simulink library "Lib_Piccolo"  (R2018b)
settings: Solver=VariableStepAuto  StartTime=0.0  StopTime=10.0  RelTol=1e-3
values from neighbouring files (symbols this model uses):
  AccelErrInt2Brakes = 0.15    [SimulationControlConfig16P.m]    (also in SimulationControlConfig16P_LEGACY.m; SimulationControlConfigTAILLESS.m = 0.2; SimulationControlConfigUTAIL.m = 0.2)
  AileronMax = 25    [SimulationControlConfig16P.m]    (also in SimulationControlConfig16P_LEGACY.m; SimulationControlConfigTAILLESS.m; SimulationControlConfigUTAIL.m)
  AileronPower = 0.00268    [SimulationControlConfig16P.m]    (also in SimulationControlConfig16P_LEGACY.m; SimulationControlConfigTAILLESS.m; SimulationControlConfigUTAIL.m)
  AileronSurfaceMax = 45    [SimulationControlConfig16P.m]    (also in SimulationControlConfig16P_LEGACY.m)
  AileronTrim = 0    [SimulationControlConfig16P.m]    (also in SimulationControlConfig16P_LEGACY.m; SimulationControlConfigTAILLESS.m; SimulationControlConfigUTAIL.m)
  Alt = 1000 + TerrainHeight    [SimulationStateConfig.m]
  AltCruise_m = testPlans(testIndx).terrainElevation * 0.3048 + 200    [SimulationControlConfig16P.m]    (also in SimulationControlConfigTAILLESS.m = 1083; SimulationControlConfigUTAIL.m = testPlans(testIndx).terrainElevation * 0.3048 + 152)
  AltitudeRate2PitchCmdIntegratorInit = 0.1    [SimulationControlPre.m]
  AltMax = 10000    [SimulationControlConfig16P.m]    (also in SimulationControlConfig16P_LEGACY.m; SimulationControlConfigTAILLESS.m; SimulationControlConfigUTAIL.m)
  AltMaxAccel = 1.25    [SimulationControlConfig16P.m]    (also in SimulationControlConfig16P_LEGACY.m = 0.9; SimulationControlConfigTAILLESS.m = 1.7; SimulationControlConfigUTAIL.m = 2)
  AltMin = 0    [SimulationControlConfig16P.m]    (also in SimulationControlConfig16P_LEGACY.m; SimulationControlConfigTAILLESS.m; SimulationControlConfigUTAIL.m)
  AltRateCmd2Pitch = 0.50    (= 0.5)    [SimulationControlConfig16P.m]    (also in SimulationControlConfig16P_LEGACY.m = 0.6; SimulationControlConfigTAILLESS.m = 0.2; SimulationControlConfigUTAIL.m = 0.3)
  AltRateError2Pitch = 0.40    (= 0.4)    [SimulationControlConfig16P.m]    (also in SimulationControlConfig16P_LEGACY.m; SimulationControlConfigTAILLESS.m = 0.55; SimulationControlConfigUTAIL.m = 0.55)
  AltRateErrorInt2Pitch = 0.50    (= 0.5)    [SimulationControlConfig16P.m]    (also in SimulationControlConfig16P_LEGACY.m = 0.45; SimulationControlConfigTAILLESS.m; SimulationControlConfigUTAIL.m = 0.75)
  AltRateLpfCutOff = 3    [SimulationControlConfig16P.m]    (also in SimulationControlConfig16P_LEGACY.m; SimulationControlConfigTAILLESS.m = 2; SimulationControlConfigUTAIL.m = 2)
  AutoNosegear2Rudder = 26    [SimulationControlConfig16P.m]    (also in SimulationControlConfig16P_LEGACY.m; SimulationControlConfigTAILLESS.m = 25.2; SimulationControlConfigUTAIL.m = 14)
  b = 5.54    [SimulationControlConfig16P.m]    (also in SimulationControlConfig16P_LEGACY.m; SimulationControlConfigTAILLESS.m = 2.37; SimulationControlConfigUTAIL.m = 2.37)
  Bank2AileronIntegratorInit = 0    [SimulationControlPre.m]
  BankMax_User = BankMax_User/180*pi    (= 0.523598775598)    [SimulationControlConfig16P.m]    (also in SimulationControlConfig16P_LEGACY.m; SimulationControlConfigTAILLESS.m = 0.610865238198; SimulationControlConfigUTAIL.m = 0.628318530718)
  baseLegFlaps = 20    [SimulationControlConfig16P.m]    (also in SimulationControlConfig16P_LEGACY.m = 0; SimulationControlConfigTAILLESS.m = 15; SimulationControlConfigUTAIL.m = 10)
  C = GeneticOpt.C    [SimulationCostFunction.m]
  c = Sw/b    (= 0.841696750903)    [SimulationControlConfig16P.m]    (also in SimulationControlConfig16P_LEGACY.m; SimulationControlConfigTAILLESS.m = 0.354008438819; SimulationControlConfigUTAIL.m = 0.354008438819)
  cell2WheelFactorMG = 5.98    [SimulationSensorConfig16P_LEGACY.m]
  cell2WheelFactorNG = 1    [SimulationSensorConfig16P_LEGACY.m]
  cellSatMaxMG = 15000    [SimulationSensorConfig16P.m]    (also in SimulationSensorConfig16P_LEGACY.m; SimulationSensorConfigTAILLESS7P.m; SimulationSensorConfigUTAIL7P.m)
  cellSatMaxNG = 1000    [SimulationSensorConfig16P.m]    (also in SimulationSensorConfig16P_LEGACY.m; SimulationSensorConfigTAILLESS7P.m; SimulationSensorConfigUTAIL7P.m)
  cellSatMinMG = -15000    [SimulationSensorConfig16P.m]    (also in SimulationSensorConfig16P_LEGACY.m; SimulationSensorConfigTAILLESS7P.m; SimulationSensorConfigUTAIL7P.m)
  cellSatMinNG = -1000    [SimulationSensorConfig16P.m]    (also in SimulationSensorConfig16P_LEGACY.m; SimulationSensorConfigTAILLESS7P.m; SimulationSensorConfigUTAIL7P.m)
  CL_Limit = CL_Max    (= 0.54)    [SimulationControlConfig16P.m]    (also in SimulationControlConfig16P_LEGACY.m; SimulationControlConfigTAILLESS.m; SimulationControlConfigUTAIL.m = 0.53)
  CL_Max = 0.54    [SimulationControlConfig16P.m]    (also in SimulationControlConfig16P_LEGACY.m; SimulationControlConfigTAILLESS.m; SimulationControlConfigUTAIL.m = 0.53)
  CL_Max_Nom = 0.465    [SimulationControlConfig16P.m]    (also in SimulationControlConfig16P_LEGACY.m; SimulationControlConfigTAILLESS.m = 0.39; SimulationControlConfigUTAIL.m)
  CL_Min = 0    [SimulationControlConfig16P.m]    (also in SimulationControlConfig16P_LEGACY.m; SimulationControlConfigTAILLESS.m; SimulationControlConfigUTAIL.m)
  ClimbMaxFraction = 0.35    [SimulationControlConfig16P.m]    (also in SimulationControlConfig16P_LEGACY.m = 0.24; SimulationControlConfigTAILLESS.m = 0.19; SimulationControlConfigUTAIL.m = 0.21)
  ClimboutMaxBank = 7.0    (= 7)    [SimulationControlConfig16P.m]    (also in SimulationControlConfig16P_LEGACY.m; SimulationControlConfigTAILLESS.m = 5; SimulationControlConfigUTAIL.m)
  ClimboutTimer = 7.0    (= 7)    [SimulationControlConfig16P.m]    (also in SimulationControlConfig16P_LEGACY.m; SimulationControlConfigTAILLESS.m; SimulationControlConfigUTAIL.m)
  dCl_per_dFlap = 0.005581818    [SimulationControlConfig16P.m]    (also in SimulationControlConfig16P_LEGACY.m = 0; SimulationControlConfigTAILLESS.m = 0; SimulationControlConfigUTAIL.m = 0)
  DecelerationCmd = 3.1    [SimulationControlConfig16P.m]    (also in SimulationControlConfig16P_LEGACY.m; SimulationControlConfigTAILLESS.m = 0.1; SimulationControlConfigUTAIL.m = 0.1)
  DeRotateLogicEndTimer = abs((NoseDownLimit_Deg-1)/DeRotateRamp_Dps)    [SimulationControlConfig16P.m]    (also in SimulationControlConfig16P_LEGACY.m; SimulationControlConfigTAILLESS.m; SimulationControlConfigUTAIL.m)
  DeRotateLogicHoldNoseUpTimer = 0.1    [SimulationControlConfig16P.m]    (also in SimulationControlConfig16P_LEGACY.m; SimulationControlConfigTAILLESS.m; SimulationControlConfigUTAIL.m)
  DeRotateLogicTimerTimeout = 2    [SimulationControlConfig16P.m]    (also in SimulationControlConfig16P_LEGACY.m; SimulationControlConfigTAILLESS.m; SimulationControlConfigUTAIL.m)
  DeRotateLowerCmdSaturation = 0    [SimulationControlConfig16P.m]    (also in SimulationControlConfig16P_LEGACY.m; SimulationControlConfigTAILLESS.m; SimulationControlConfigUTAIL.m)
  DeRotateRamp_Dps = 3    [SimulationControlConfig16P.m]    (also in SimulationControlConfig16P_LEGACY.m; SimulationControlConfigTAILLESS.m = 8; SimulationControlConfigUTAIL.m = 8)
  DeRotateUpperCmdSaturation = 7    [SimulationControlConfig16P.m]    (also in SimulationControlConfig16P_LEGACY.m; SimulationControlConfigTAILLESS.m; SimulationControlConfigUTAIL.m)
  DescentMaxFraction = 0.22    [SimulationControlConfig16P.m]    (also in SimulationControlConfig16P_LEGACY.m = 0.2; SimulationControlConfigTAILLESS.m = 0.17; SimulationControlConfigUTAIL.m = 0.17)
  DesktopSimTerrainOffset_m = 0.406    [SimulationAircraftConfig.m]
  downwindFlaps = 0    [SimulationControlConfig16P.m]    (also in SimulationControlConfig16P_LEGACY.m; SimulationControlConfigTAILLESS.m; SimulationControlConfigUTAIL.m)
  DP_init = 0.5*1.225*V_init^2    [SimulationControlConfig16P.m]    (also in SimulationControlConfig16P_LEGACY.m; SimulationControlConfigTAILLESS.m; SimulationControlConfigUTAIL.m)
  dscNoiseMG = 1    [SimulationSensorConfig16P_LEGACY.m]
  dscNoiseNG = 0.25    [SimulationSensorConfig16P_LEGACY.m]
  DSCnumBits = 24    [SimulationSensorConfig16P.m]    (also in SimulationSensorConfig16P_LEGACY.m; SimulationSensorConfigTAILLESS7P.m; SimulationSensorConfigUTAIL7P.m)
  DSCRangeMaxMG = 15000    [SimulationSensorConfig16P.m]    (also in SimulationSensorConfig16P_LEGACY.m; SimulationSensorConfigTAILLESS7P.m; SimulationSensorConfigUTAIL7P.m)
  DSCRangeMaxNG = 1000    [SimulationSensorConfig16P.m]    (also in SimulationSensorConfig16P_LEGACY.m; SimulationSensorConfigTAILLESS7P.m; SimulationSensorConfigUTAIL7P.m)
  DSCRangeMinMG = -15000    [SimulationSensorConfig16P.m]    (also in SimulationSensorConfig16P_LEGACY.m; SimulationSensorConfigTAILLESS7P.m; SimulationSensorConfigUTAIL7P.m)
  DSCRangeMinNG = -1000    [SimulationSensorConfig16P.m]    (also in SimulationSensorConfig16P_LEGACY.m; SimulationSensorConfigTAILLESS7P.m; SimulationSensorConfigUTAIL7P.m)
  dt = DLLSim.dt    [SimulationTimeStep.m]    (also in SimulationTrim.m = 0.02)
  EarlyTouchdownThreshold = 3.0    (= 3)    [SimulationControlConfig16P.m]    (also in SimulationControlConfig16P_LEGACY.m; SimulationControlConfigTAILLESS.m = 2.2; SimulationControlConfigUTAIL.m = 2.5)
  ElevatorDeflectionRate = 15    [SimulationControlConfig16P.m]    (also in SimulationControlConfig16P_LEGACY.m = 12; SimulationControlConfigTAILLESS.m = 10; SimulationControlConfigUTAIL.m = 12)
  ElevatorMax = 25    [SimulationControlConfig16P.m]    (also in SimulationControlConfig16P_LEGACY.m; SimulationControlConfigTAILLESS.m; SimulationControlConfigUTAIL.m)
  ElevatorPower = -0.002209    [SimulationControlConfig16P.m]    (also in SimulationControlConfig16P_LEGACY.m; SimulationControlConfigTAILLESS.m = -0.002956; SimulationControlConfigUTAIL.m = -0.00205983)
  ElevatorTrim = -3.5    [SimulationControlConfig16P.m]    (also in SimulationControlConfig16P_LEGACY.m; SimulationControlConfigTAILLESS.m = -6; SimulationControlConfigUTAIL.m = -8)
  elevonBias = 0    [SimulationControlConfig16P.m]    (also in SimulationControlConfig16P_LEGACY.m; SimulationControlConfigTAILLESS.m; SimulationControlConfigUTAIL.m)
  Enable_TAS_Protection = 0    [SimulationControlConfig16P.m]    (also in SimulationControlConfig16P_LEGACY.m; SimulationControlConfigTAILLESS.m; SimulationControlConfigUTAIL.m)
  EnableCrossTrackAbort = 1    [SimulationControlConfig16P.m]    (also in SimulationControlConfigTAILLESS.m; SimulationControlConfigUTAIL.m)
  EnergyBandwidth = 0.02    [SimulationControlConfig16P.m]    (also in SimulationControlConfig16P_LEGACY.m; SimulationControlConfigTAILLESS.m = 0.06; SimulationControlConfigUTAIL.m = 0.06)
  EngineLhFuelCut = 0    [SimulationAircraftConfig.m]
  EngineRhFuelCut = 0    [SimulationAircraftConfig.m]
  FastThrottleRate = 0.075    [SimulationControlConfig16P.m]    (also in SimulationControlConfig16P_LEGACY.m = 0.05; SimulationControlConfigTAILLESS.m = 0.1; SimulationControlConfigUTAIL.m = 0.1)
  FilterWarmUpTime = 2    [SimulationSensorConfig16P.m]    (also in SimulationSensorConfig16P_LEGACY.m; SimulationSensorConfigTAILLESS7P.m; SimulationSensorConfigUTAIL7P.m)
  finalApproachFlaps = 20    [SimulationControlConfig16P.m]    (also in SimulationControlConfig16P_LEGACY.m = 0; SimulationControlConfigTAILLESS.m = 22; SimulationControlConfigUTAIL.m = 10)
  FinalDescentSlope_Deg = testPlans(testIndx).descentSlope    [SimulationControlConfig16P.m]    (also in SimulationControlConfig16P_LEGACY.m; SimulationControlConfigTAILLESS.m; SimulationControlConfigUTAIL.m)
  flapMax = 0    [SimulationControlConfig16P.m]    (also in SimulationControlConfig16P_LEGACY.m; SimulationControlConfigTAILLESS.m; SimulationControlConfigUTAIL.m)
  flapRate = 7.5    [SimulationControlConfig16P.m]    (also in SimulationControlConfig16P_LEGACY.m; SimulationControlConfigTAILLESS.m = 6.6; SimulationControlConfigUTAIL.m)
  FlareHeight = 5    [SimulationControlConfig16P.m]    (also in SimulationControlConfig16P_LEGACY.m = 4.8; SimulationControlConfigTAILLESS.m = 2.5; SimulationControlConfigUTAIL.m = 2)
  FlareVerticalRate_mps = -0.4    [SimulationControlConfig16P.m]    (also in SimulationControlConfig16P_LEGACY.m = -0.5; SimulationControlConfigTAILLESS.m = -0.15; SimulationControlConfigUTAIL.m = -0.15)
  Fp_Aileron = 0.55*2*pi*RollRateLpfCutoff*dt    [SimulationControlConfig16P.m]    (also in SimulationControlConfig16P_LEGACY.m; SimulationControlConfigTAILLESS.m; SimulationControlConfigUTAIL.m)
  Fp_Alt = 0.55*AltBandwidth    (= 0.099)    [SimulationControlConfig16P.m]    (also in SimulationControlConfig16P_LEGACY.m; SimulationControlConfigTAILLESS.m = 0.587477826221; SimulationControlConfigUTAIL.m = 0.69115038379)
  Fp_AltRate = 0.55*2*pi*AltRateLpfCutOff*dt    [SimulationControlConfig16P.m]    (also in SimulationControlConfig16P_LEGACY.m; SimulationControlConfigTAILLESS.m; SimulationControlConfigUTAIL.m)
  Fp_Elevator = 0.55*2*pi*PitchRateLpfCutoff*dt    [SimulationControlConfig16P.m]    (also in SimulationControlConfig16P_LEGACY.m; SimulationControlConfigTAILLESS.m; SimulationControlConfigUTAIL.m)
  Fp_Energy = 0.55*2*pi*EnergyBandwidth    (= 0.069115038379)    [SimulationControlConfig16P.m]    (also in SimulationControlConfig16P_LEGACY.m; SimulationControlConfigTAILLESS.m = 0.207345115137; SimulationControlConfigUTAIL.m = 0.207345115137)
  Fp_Energy2 = 0.55*2*pi*EnergyBandwidth*dt    [SimulationControlConfig16P.m]    (also in SimulationControlConfig16P_LEGACY.m; SimulationControlConfigTAILLESS.m; SimulationControlConfigUTAIL.m)
  Fp_Pitch = 0.55*2*pi*PitchBandwidth    (= 2.76460153516)    [SimulationControlConfig16P.m]    (also in SimulationControlConfig16P_LEGACY.m = 3.11017672705; SimulationControlConfigTAILLESS.m = 3.80132711084; SimulationControlConfigUTAIL.m = 2.41902634326)
  Fp_Pitch_2 = 0.55*2*pi*PitchBandwidth*dt    [SimulationControlConfig16P.m]    (also in SimulationControlConfig16P_LEGACY.m; SimulationControlConfigTAILLESS.m; SimulationControlConfigUTAIL.m)
  Fp_Roll = RollBandwidth^2    (= 1)    [SimulationControlConfig16P.m]    (also in SimulationControlConfig16P_LEGACY.m = 1.44; SimulationControlConfigTAILLESS.m; SimulationControlConfigUTAIL.m)
  Fp_Rudder = 0.55*2*pi*YawRateLpfCutoff*dt    [SimulationControlConfig16P.m]    (also in SimulationControlConfig16P_LEGACY.m; SimulationControlConfigTAILLESS.m; SimulationControlConfigUTAIL.m)
  Fp_TAS = 0.55*2*pi*TASBandwidth    (= 0.103672557568)    [SimulationControlConfig16P.m]    (also in SimulationControlConfig16P_LEGACY.m; SimulationControlConfigTAILLESS.m = 0.172787595947; SimulationControlConfigUTAIL.m = 0.172787595947)
  Fp_TAS_Filter = 2*pi*TasLpfCutoff*dt    [SimulationControlConfig16P.m]    (also in SimulationControlConfig16P_LEGACY.m; SimulationControlConfigTAILLESS.m; SimulationControlConfigUTAIL.m)
  Fp_Turn = 0.55*2*pi*TurnErrLPFcutoff    (= 0.0345575191895)    [SimulationControlConfig16P.m]    (also in SimulationControlConfig16P_LEGACY.m; SimulationControlConfigTAILLESS.m = 0.172787595947; SimulationControlConfigUTAIL.m = 0.172787595947)
  Fp_TurnDerr = 0.55*2*pi*TurnDerivativeLPFcutoff    (= 0.0345575191895)    [SimulationControlConfig16P.m]    (also in SimulationControlConfig16P_LEGACY.m; SimulationControlConfigTAILLESS.m = 0.172787595947; SimulationControlConfigUTAIL.m = 0.172787595947)
  FTV = 3    [SimulationAircraftConfig.m]
  ftvStaticPositionError = 1/1.18    (= 0.847457627119)    [SimulationSensorConfig16P.m]    (also in SimulationSensorConfig16P_LEGACY.m; SimulationSensorConfigTAILLESS7P.m = 1; SimulationSensorConfigUTAIL7P.m = 1)
  g = 9.81    [SimulationStateConfig.m]
  GustSpd_Kts = testPlans(testIndx).gustSpd    [SimulationStateConfig.m]
  GustTriggerVal = testPlans(testIndx).gustTriggerVal    [SimulationStateConfig.m]
  HeadingErr2TurnRate = 0.5    [SimulationControlConfig16P.m]    (also in SimulationControlConfig16P_LEGACY.m; SimulationControlConfigTAILLESS.m; SimulationControlConfigUTAIL.m)
  HeadingErrDer2TurnRate = 0.3    [SimulationControlConfig16P.m]    (also in SimulationControlConfig16P_LEGACY.m; SimulationControlConfigTAILLESS.m; SimulationControlConfigUTAIL.m)
  IASbounce = IASstall*0.8    [SimulationControlPre.m]
  IAScruiseCMD = sqrt(2*m*9.81/(1.225*Sw*CL_cruise))    [SimulationControlConfig16P.m]    (also in SimulationControlConfig16P_LEGACY.m; SimulationControlConfigTAILLESS.m; SimulationControlConfigUTAIL.m)
  IASfinalCMD = 1.12 * IASmin    [SimulationControlConfig16P.m]    (also in SimulationControlConfig16P_LEGACY.m = 1.10 * IASmin; SimulationControlConfigTAILLESS.m = 1.10 * IASmin; SimulationControlConfigUTAIL.m = 1.15 * IASmin)
  IASflareCMD = IASstall    [SimulationControlConfig16P.m]    (also in SimulationControlConfig16P_LEGACY.m; SimulationControlConfigTAILLESS.m; SimulationControlConfigUTAIL.m)
  IASmax = 64    [SimulationControlConfig16P.m]    (also in SimulationControlConfig16P_LEGACY.m = 46; SimulationControlConfigTAILLESS.m = 38.58; SimulationControlConfigUTAIL.m = 35)
  IASmin = sqrt(2*m*9.81/(1.225*Sw*0.9*CL_Max_Nom))    [SimulationControlConfig16P.m]    (also in SimulationControlConfig16P_LEGACY.m; SimulationControlConfigTAILLESS.m; SimulationControlConfigUTAIL.m)
  IASshortCMD = IASstall    [SimulationControlConfig16P.m]    (also in SimulationControlConfig16P_LEGACY.m; SimulationControlConfigTAILLESS.m; SimulationControlConfigUTAIL.m)
  IASstall = sqrt(2*m*9.81/(1.225*Sw*CL_Max))    [SimulationControlConfig16P.m]    (also in SimulationControlConfig16P_LEGACY.m; SimulationControlConfigTAILLESS.m; SimulationControlConfigUTAIL.m)
  inFlight = 1    [SimulationControlConfig16P.m]    (also in SimulationControlConfigTAILLESS.m; SimulationControlConfigUTAIL.m)
  JetCatOffset = 5    [SimulationControlConfig16P.m]    (also in SimulationControlConfig16P_LEGACY.m)
  LaunchRollingElevator = -1.5    [SimulationControlConfig16P.m]    (also in SimulationControlConfig16P_LEGACY.m; SimulationControlConfigTAILLESS.m = 1; SimulationControlConfigUTAIL.m = 1)
  ldg_NosegearMax = 10    [SimulationControlConfig16P.m]    (also in SimulationControlConfig16P_LEGACY.m; SimulationControlConfigTAILLESS.m; SimulationControlConfigUTAIL.m)
  ldg_TrackVyErrInt2Nosegear = 0.1250    (= 0.125)    [SimulationControlConfig16P.m]    (also in SimulationControlConfig16P_LEGACY.m; SimulationControlConfigTAILLESS.m = 0.00714285714286; SimulationControlConfigUTAIL.m = 0.00714285714286)
  ldg_TrackVyErrPro2Nosegear = 0.35    [SimulationControlConfig16P.m]    (also in SimulationControlConfig16P_LEGACY.m; SimulationControlConfigTAILLESS.m = 0.0546666666667; SimulationControlConfigUTAIL.m = 0.0546666666667)
  ldg_TrackY2Vy = 0.07    [SimulationControlConfig16P.m]    (also in SimulationControlConfig16P_LEGACY.m; SimulationControlConfigTAILLESS.m = 0.17; SimulationControlConfigUTAIL.m = 0.17)
  ldg_Vy2NosegearScalingPower = 1.075    [SimulationControlConfig16P.m]    (also in SimulationControlConfig16P_LEGACY.m; SimulationControlConfigTAILLESS.m = 0.6; SimulationControlConfigUTAIL.m = 0.5)
  ldg_Y2VyScalingPower = 0.175    [SimulationControlConfig16P.m]    (also in SimulationControlConfig16P_LEGACY.m; SimulationControlConfigTAILLESS.m = 0; SimulationControlConfigUTAIL.m = 0)
  ldg_YawRate2Nosegear = 0.175    [SimulationControlConfig16P.m]    (also in SimulationControlConfig16P_LEGACY.m; SimulationControlConfigTAILLESS.m = 0.065; SimulationControlConfigUTAIL.m = 0.065)
  LiftSlope = 0.064285    [SimulationControlConfig16P.m]    (also in SimulationControlConfig16P_LEGACY.m; SimulationControlConfigTAILLESS.m = 0.058631; SimulationControlConfigUTAIL.m)
  LPFaileronInit = 0    [SimulationControlPre.m]
  LPFclestInit = 0    [SimulationControlPre.m]
  LPFenergyFFInit = 0    [SimulationControlPre.m]
  LPFtasInit = V_init + 2    [SimulationControlPre.m]
  LPFthrottleInit = ThrottleTrim    [SimulationControlPre.m]
  LPFturnErrInit = 0    [SimulationControlPre.m]
  ... (+115 more)
undefined symbols (not defined in the file or in its folder): abortFlag, alphaHPF, apmDelay, BRWNOUT, CRAWOR, CRAWUR, DiscIntNeverNeededParam, DLLSim, DLLSimStep, ECOMOR, ECOMUR, Fp_Tas, GustTrigger_HeightAgl_m, IPSTAT, LCINTEG, Ldg_Persist_Time, LOWER_FLAGS, MSG_ENABLE, NoiseStd, OLDVAL, OVERRIDE_ENABLE, OVERRIDE_VALUE, REBOOT, reversionEnable, revIASMax, revIASMin, revPitchMax, revPitchMin, revPitchRateMax, revRollMax, revRollRateMax, SAMPLE, SCALON, SensorModel, sigbuilder_block, Sim_Vx, Sim_Vy, Sim_Vz, Sim_Xpos, Sim_Ypos, Sim_Zpos, SYSOR, SYSUR, TARE, TEMPOR, TEMPUR, testIndx, testPlan, testPlans, Trim_piccoloInCmd, Trim_REFSI_FD_IN_nmodeCgShifterCmd_Ft, Trim_REFSI_FD_IN_nmodeFlapLhIBCmd_Deg, Trim_REFSI_FD_IN_nmodeFlapLhOBCmd_Deg, Trim_REFSI_FD_IN_nmodeFlapRhIBCmd_Deg, Trim_REFSI_FD_IN_nmodeFlapRhOBCmd_Deg, Trim_REFSI_FD_IN_nmodeSlatLhCmd_Deg, Trim_REFSI_FD_IN_nmodeSlatRhCmd_Deg, Trim_REFSI_FD_IN_nmodeSplrLhInbdCmd_Deg, Trim_REFSI_FD_IN_nmodeSplrLhOutbdCmd_Deg ... (+5)
libraries: simulink x866, aerolibconvert2 x60, $bdroot x52, aerolibatmos2 x5, dspswit3 x5, simulink_extras x4, dsparch4 x2, Lib_Piccolo_Alt x2, eeGeneralControl x1, dspindex x1
(part 21 of 44)

== system Lib_Piccolo/Ground Detection Systems/WoW Wrapper/Variant Subsystem ==
  note: 16 - Logic derived from LOAD2, with key changes:
      | - Saturation on inputs to filter to prevent 'wind-up'
      | - Fix to signal probe location used to drive one-wheel and persistence chain (this is a change from LOAD14)
      |
      | NOTE - this variant of the model has updates & simplifications to model elements upstream of the K2 and correct representation of DSC resolution. Not propagated to previous variants!
  note: 1) Add Subsystem or Model blocks as valid variant choices.
      | 2) You cannot connect blocks at this level. At simulation, connectivity is automatically
      | determined, based on the active variant and port name matching.
  note: 18 - Core logic & modelling is matched to 16 , with updates to accomodate landing with single-wheel DSC failures.
  note: 20 - Detection logic is that of 16 with addition of single-wheel failure handling . System further developed in Simulink for test & code-generation capability.
  Piccolo_AP_Mode : Inport
  WoW_Bus_In : Inport  Port=2
  Load Cell WoW Model 1 : Subsystem  VariantControl="SensorModel.WOW.Cell.Variant==\"LOAD1\""  mask{Ldg_Persist_Time=SensorModel.WOW.Cell.persistanceTime_s, Ldg_Latch_Time_P=SensorModel.WOW.Cell.longLatchTime_s, Ldg_Latch_Time_S=SensorModel.WOW.Cell.shortLatchTime_s, Ldg_Load_Thresh_Upper=SensorModel.WOW.Cell.loadThresholdUpper_N, Ldg_Load_Thresh_Lower=SensorModel.WOW.Cell.loadThresholdLower_N, TO_Persist_Time=SensorModel.WOW.Cell.TO_persistanceTime_s, TO_Latch_Time=SensorModel.WOW.Cell.TO_latchTime_s, TO_Load_Thresh=SensorModel.WOW.Cell.TO_loadThreshold_N, DSCnumBits=24, numBits=16, satMaxMG=15000, satMinMG=-300, dscNoiseMG=1, DSCRangeMaxMG=15000, DSCRangeMinMG=-15000, satMaxNG=1000, satMinNG=-250, dscNoiseNG=0.25, DSCRangeMaxNG=1000, DSCRangeMinNG=-1000, cellSatMaxMG=15000, cellSatMinMG=-15000, cell2WheelFactorMG=5.98, cellSatMaxNG=1000, cellSatMinNG=-1000, cell2WheelFactorNG=1}
      mask prompts: Ldg_Persist_Time "Landing Persistance Time [s]"; Ldg_Latch_Time_P "Primary Landing Latch Time [s]"; Ldg_Latch_Time_S "Secondary Landing Latch Time [s]"; Ldg_Load_Thresh_Upper "Landing Load Threshold Upper [N]"; Ldg_Load_Thresh_Lower "Landing Load Threshold Lower [N]"; TO_Persist_Time "Take Off Persistance Time [s]"; TO_Latch_Time "Take Off Latch Time [s]"; TO_Load_Thresh "Take Off Load Threshold  [N]"; DSCnumBits "DSC Encoded Resolution [num bits]"; numBits "CANBridge Encoded Resolution [num bits]"; satMaxMG "Main Gear CANBridge Saturation Max [N]"; satMinMG "Main Gear CANBridge Saturation Min [N]"; dscNoiseMG "Main Gear DSC Noise Level pk-pk [N]"; DSCRangeMaxMG "Main Gear DSC Range Max [N]"; DSCRangeMinMG "Main Gear DSC Range Min [N]"; satMaxNG "Nose Gear CANBridge Saturation Max [N]"; satMinNG "Nose Gear CANBridge Saturation Min [N]"; dscNoiseNG "Nose Gear DSC Noise Level pk-pk [N]"; DSCRangeMaxNG "Nose Gear DSC Range Max [N]"; DSCRangeMinNG "Nose Gear DSC Range Min [N]"; cellSatMaxMG "Main Gear Cell Saturation Max [N]"; cellSatMinMG "Main Gear Cell Saturation Min [N]"; cell2WheelFactorMG "Main Gear Cell to Wheel Load Scale Factor"; cellSatMaxNG "Nose Gear Cell Saturation Max [N]"; cellSatMinNG "Nose Gear Cell Saturation Min [N]"; cell2WheelFactorNG "Nose Gear Cell to Wheel Load Scale Factor"
      mask DialogControl DescGroupVar Prompt: Full model of load-cell based weight-on-wheels system.
      mask DialogControl LogicGroupVar Prompt: Logic Configuration
      mask DialogControl DataGroupVar Prompt: Data Acquisition
      mask DialogControl Container5 Prompt: MG
      mask DialogControl Container6 Prompt: NG
      mask DialogControl ParamGroupVar Prompt: Physical Parameters
      mask DialogControl Container8 Prompt: MG
      mask DialogControl Container9 Prompt: NG
  Load Cell WoW Model 1 16P5 AsFlown 2022 : Subsystem  VariantControl="SensorModel.WOW.Cell.Variant==\"LOAD1_16P5_ASFLOWN\""  mask{Ldg_Persist_Time=0.06, Ldg_Latch_Time_P=0.7, Ldg_Latch_Time_S=0.4, Ldg_Load_Thresh_Upper=85, Ldg_Load_Thresh_Lower=27, TO_Persist_Time=0.02, TO_Latch_Time=0.5, TO_Load_Thresh=275, DSCnumBits=24, numBits=16, satMaxMG=15000, satMinMG=-300, dscNoiseMG=1, DSCRangeMaxMG=15000, DSCRangeMinMG=-15000, satMaxNG=1000, satMinNG=-250, dscNoiseNG=0.25, DSCRangeMaxNG=1000, DSCRangeMinNG=-1000, cellSatMaxMG=15000, cellSatMinMG=-15000, cell2WheelFactorMG=5.98, cellSatMaxNG=1000, cellSatMinNG=-1000, cell2WheelFactorNG=1}
      mask prompts: Ldg_Persist_Time "Landing Persistance Time [s]"; Ldg_Latch_Time_P "Primary Landing Latch Time [s]"; Ldg_Latch_Time_S "Secondary Landing Latch Time [s]"; Ldg_Load_Thresh_Upper "Landing Load Threshold Upper [N]"; Ldg_Load_Thresh_Lower "Landing Load Threshold Lower [N]"; TO_Persist_Time "Take Off Persistance Time [s]"; TO_Latch_Time "Take Off Latch Time [s]"; TO_Load_Thresh "Take Off Load Threshold  [N]"; DSCnumBits "DSC Encoded Resolution [num bits]"; numBits "CANBridge Encoded Resolution [num bits]"; satMaxMG "Main Gear CANBridge Saturation Max [N]"; satMinMG "Main Gear CANBridge Saturation Min [N]"; dscNoiseMG "Main Gear DSC Noise Level pk-pk [N]"; DSCRangeMaxMG "Main Gear DSC Range Max [N]"; DSCRangeMinMG "Main Gear DSC Range Min [N]"; satMaxNG "Nose Gear CANBridge Saturation Max [N]"; satMinNG "Nose Gear CANBridge Saturation Min [N]"; dscNoiseNG "Nose Gear DSC Noise Level pk-pk [N]"; DSCRangeMaxNG "Nose Gear DSC Range Max [N]"; DSCRangeMinNG "Nose Gear DSC Range Min [N]"; cellSatMaxMG "Main Gear Cell Saturation Max [N]"; cellSatMinMG "Main Gear Cell Saturation Min [N]"; cell2WheelFactorMG "Main Gear Cell to Wheel Load Scale Factor"; cellSatMaxNG "Nose Gear Cell Saturation Max [N]"; cellSatMinNG "Nose Gear Cell Saturation Min [N]"; cell2WheelFactorNG "Nose Gear Cell to Wheel Load Scale Factor"
      mask DialogControl DescGroupVar Prompt: Full model of load-cell based weight-on-wheels system.
      mask DialogControl LogicGroupVar Prompt: Logic Configuration
      mask DialogControl DataGroupVar Prompt: Data Acquisition
      mask DialogControl Container5 Prompt: MG
      mask DialogControl Container6 Prompt: NG
      mask DialogControl ParamGroupVar Prompt: Physical Parameters
      mask DialogControl Container8 Prompt: MG
      mask DialogControl Container9 Prompt: NG
  Load Cell WoW Model 1 7P AsFlown : Subsystem  VariantControl="SensorModel.WOW.Cell.Variant==\"LOAD1_7P_ASFLOWN\""  mask{Ldg_Persist_Time=0.06, Ldg_Latch_Time_P=0.5, Ldg_Latch_Time_S=0.5, Ldg_Load_Thresh_Upper=10, Ldg_Load_Thresh_Lower=3.5, TO_Persist_Time=0.02, TO_Latch_Time=0.5, TO_Load_Thresh=21.15, DSCnumBits=24, numBits=16, satMaxMG=15000, satMinMG=-300, dscNoiseMG=1, DSCRangeMaxMG=15000, DSCRangeMinMG=-15000, satMaxNG=1000, satMinNG=-250, dscNoiseNG=0.25, DSCRangeMaxNG=1000, DSCRangeMinNG=-1000, cellSatMaxMG=15000, cellSatMinMG=-15000, cell2WheelFactorMG=5.98, cellSatMaxNG=1000, cellSatMinNG=-1000, cell2WheelFactorNG=1}
      mask prompts: Ldg_Persist_Time "Landing Persistance Time [s]"; Ldg_Latch_Time_P "Primary Landing Latch Time [s]"; Ldg_Latch_Time_S "Secondary Landing Latch Time [s]"; Ldg_Load_Thresh_Upper "Landing Load Threshold Upper [N]"; Ldg_Load_Thresh_Lower "Landing Load Threshold Lower [N]"; TO_Persist_Time "Take Off Persistance Time [s]"; TO_Latch_Time "Take Off Latch Time [s]"; TO_Load_Thresh "Take Off Load Threshold  [N]"; DSCnumBits "DSC Encoded Resolution [num bits]"; numBits "CANBridge Encoded Resolution [num bits]"; satMaxMG "Main Gear CANBridge Saturation Max [N]"; satMinMG "Main Gear CANBridge Saturation Min [N]"; dscNoiseMG "Main Gear DSC Noise Level pk-pk [N]"; DSCRangeMaxMG "Main Gear DSC Range Max [N]"; DSCRangeMinMG "Main Gear DSC Range Min [N]"; satMaxNG "Nose Gear CANBridge Saturation Max [N]"; satMinNG "Nose Gear CANBridge Saturation Min [N]"; dscNoiseNG "Nose Gear DSC Noise Level pk-pk [N]"; DSCRangeMaxNG "Nose Gear DSC Range Max [N]"; DSCRangeMinNG "Nose Gear DSC Range Min [N]"; cellSatMaxMG "Main Gear Cell Saturation Max [N]"; cellSatMinMG "Main Gear Cell Saturation Min [N]"; cell2WheelFactorMG "Main Gear Cell to Wheel Load Scale Factor"; cellSatMaxNG "Nose Gear Cell Saturation Max [N]"; cellSatMinNG "Nose Gear Cell Saturation Min [N]"; cell2WheelFactorNG "Nose Gear Cell to Wheel Load Scale Factor"
      mask DialogControl DescGroupVar Prompt: Full model of load-cell based weight-on-wheels system.
      mask DialogControl LogicGroupVar Prompt: Logic Configuration
      mask DialogControl DataGroupVar Prompt: Data Acquisition
      mask DialogControl Container5 Prompt: MG
      mask DialogControl Container6 Prompt: NG
      mask DialogControl ParamGroupVar Prompt: Physical Parameters
      mask DialogControl Container8 Prompt: MG
      mask DialogControl Container9 Prompt: NG
  Load Cell WoW Model 16 : Subsystem  VariantControl="SensorModel.WOW.Cell.Variant==\"LOAD16\""
  Load Cell WoW Model 18 : Subsystem  VariantControl="SensorModel.WOW.Cell.Variant==\"LOAD18\""
  Load Cell WoW Model 20 : Subsystem  VariantControl="SensorModel.WOW.Cell.Variant==\"LOAD20\""
  WOW_Bus_Out : Outport

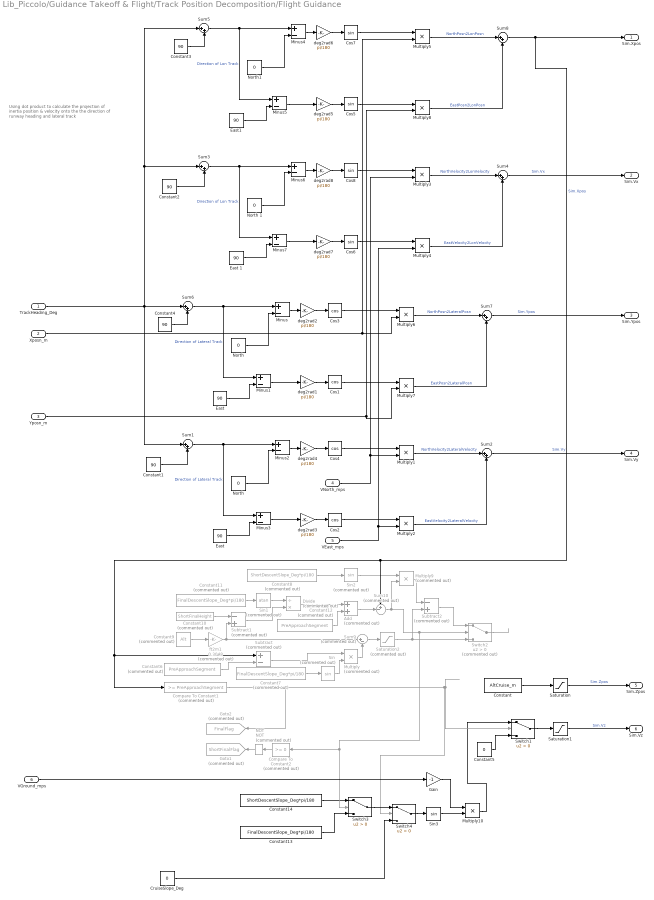
== system Lib_Piccolo/Guidance Takeoff & Flight/Track Position Decomposition/Flight Guidance ==
  note: Using dot product to calculate the projection of inertia position & velocity onto the
      | the direction of runway heading and lateral track
  TrackHeading_Deg : Inport
  Xposn_m : Inport  Port=2
  Yposn_m : Inport  Port=3
  VNorth_mps : Inport  Port=4
  VEast_mps : Inport  Port=5
  VGround_mps : Inport  Port=6
  Add : Sum  Commented=on
  Compare To Constant1 : simulink/Logic and Bit Operations/Compare To Constant  Commented=on  relop=>=  const=PreApproachSegment  OutDataTypeStr=uint8
  Compare To Constant2 : simulink/Logic and Bit Operations/Compare To Constant  Commented=on  relop=>=  const=0  OutDataTypeStr=uint8
  Constant : Constant  Value=AltCruise_m
  Constant{1..4} (4 alike) : Constant  Value=90
  Constant10 : Constant  Commented=on  Value=ShortFinalHeight
  Constant11 : Constant  Commented=on  Value=FinalDescentSlope_Deg*pi/180
  Constant12 : Constant  Commented=on  Value=PreApproachSegment
  Constant13 : Constant  Value=FinalDescentSlope_Deg*pi/180
  Constant14 : Constant  Value=ShortDescentSlope_Deg*pi/180
  Constant5 : Constant  Value=0
  Constant6 : Constant  Commented=on  Value=PreApproachSegment
  Constant7 : Constant  Commented=on  Value=FinalDescentSlope_Deg*pi/180
  Constant8 : Constant  Commented=on  Value=ShortDescentSlope_Deg*pi/180
  Constant9 : Constant  Commented=on  Value=Alt
  Cos{1..4} (4 alike) : Trigonometry  Operator=cos
  Cos{5..8} (4 alike) : Trigonometry
  CruiseSlope_Deg : Constant  Value=0
  Divide : Product  Commented=on  Inputs=/*
  East : Constant  Value=90
  "East " : Constant  Value=90
  East 1 : Constant  Value=90
  East1 : Constant  Value=90
  Gain : Gain  Gain=-1
  Goto1 : Goto  Commented=on  GotoTag=ShortFinalFlag  TagVisibility=global
  Goto2 : Goto  Commented=on  GotoTag=FinalFlag  TagVisibility=global
  Minus{,1..7} (8 alike) : Sum  Inputs=+-
  Multiply : Product  Commented=on
  Multiply{1..8,10} (9 alike) : Product
  Multiply9 : Product  Commented=on
  NOT : Logic  Commented=on  Operator=NOT  IconShape=distinctive  AllPortsSameDT=off  OutDataTypeStr=boolean
  North : Constant  Value=0
  "North " : Constant  Value=0
  North 1 : Constant  Value=0
  North1 : Constant  Value=0
  Saturation : Saturate  UpperLimit=AltMax  LowerLimit=TerrainHeight*0.3048
  Saturation1 : Saturate  UpperLimit=100  LowerLimit=-100
  Saturation2 : Saturate  Commented=on  UpperLimit=AltMax  LowerLimit=ShortFinalHeight
  Sin : Trigonometry  Commented=on
  Sin1 : Trigonometry  Commented=on  Operator=atan
  Sin2 : Trigonometry  Commented=on
  Sin3 : Trigonometry
  Subtract : Sum  Commented=on  Inputs=+-
  Subtract1 : Sum  Commented=on  Inputs=-+
  Subtract2 : Sum  Commented=on  Inputs=-+
  Sum{1..8} (8 alike) : Sum  Inputs=|++
  Sum10 : Sum  Commented=on  Inputs=+-|
  Sum9 : Sum  Commented=on  Inputs=|+-
  Switch1 : Switch  Criteria=u2 > Threshold
  Switch2 : Switch  Commented=on  Criteria=u2 > Threshold
  Switch3 : Switch  Criteria=u2 > Threshold
  Switch4 : Switch  Criteria=u2 > Threshold
  deg2rad{1..8} (8 alike) : Gain  Gain=pi/180
  ft2m1 : Gain  Commented=on  Gain=0.3048
  Sim.Xpos : Outport
  Sim.Vx : Outport  Port=2
  Sim.Ypos : Outport  Port=3
  Sim.Vy : Outport  Port=4
  Sim.Zpos : Outport  Port=5
  Sim.Vz : Outport  Port=6
  wires:
  Multiply4/1 -> Sum4/2  "EastVelocity2LonVelocity"
  VNorth_mps/1 -> Multiply3/2, Multiply1/2
  Cos2/1 -> Multiply2/1
  Constant14/1 -> Switch3/1
  Switch4/1 -> Sin3/1
  Constant9/1 -> ft2m1/1
  Minus/1 -> deg2rad2/1
  Constant6/1 -> Subtract/2
  Add/1 -> Sum10/2
  Sum9/1 -> Saturation2/1
  Cos3/1 -> Multiply6/1
  Sum4/1 -> Sim.Vx/1  "Sim.Vx"
  Sum1/1 -> Minus2/1, Minus3/1  "Direction of Lateral Track"
  deg2rad4/1 -> Cos4/1
  Sum6/1 -> Minus/1, Minus1/1  "Direction of Lateral Track"
  Constant12/1 -> Add/2
  Minus5/1 -> deg2rad5/1
  VEast_mps/1 -> Multiply4/2, Multiply2/2
  Sum10/1 -> Switch3/2, Compare To Constant2/1, Switch2/2, Multiply9/2
  Gain/1 -> Multiply10/1
  North/1 -> Minus/2
  Sum3/1 -> Minus6/1, Minus7/1  "Direction of Lon Track"
  Minus3/1 -> deg2rad3/1
  CruiseSlope_Deg/1 -> Switch4/3
  TrackHeading_Deg/1 -> Sum6/1, Sum3/1, Sum5/1, Sum1/1
  Multiply10/1 -> Switch1/1
  Multiply5/1 -> Sum8/1  "NorthPosn2LonPosn"
  Saturation2/1 -> Subtract2/2, Switch2/3
  Multiply7/1 -> Sum7/2  "EastPosn2LateralPosn"
  Multiply8/1 -> Sum8/2  "EastPosn2LonPosn"
  Minus2/1 -> deg2rad4/1
  Xposn_m/1 -> Multiply5/2, Multiply6/2
  Multiply6/1 -> Sum7/1  "NorthPosn2LateralPosn"
  Multiply/1 -> Sum9/2
  Multiply1/1 -> Sum2/1  "NorthVelocity2LateralVelocity"
  Sin2/1 -> Multiply9/1
  Constant1/1 -> Sum1/2
  NOT/1 -> Goto1/1
  Compare To Constant1/1 -> Switch4/2, Switch1/2, Goto2/1
  "North "/1 -> Minus2/2
  Multiply3/1 -> Sum4/1  "NorthVelocity2LonVelocity"
  Switch1/1 -> Saturation1/1
  Yposn_m/1 -> Multiply7/2, Multiply8/2
  Constant/1 -> Saturation/1
  ft2m1/1 -> Subtract1/2, Sum9/1
  Switch3/1 -> Switch4/1
  North 1/1 -> Minus6/2
  Subtract/1 -> Multiply/1
  Compare To Constant2/1 -> NOT/1
  deg2rad8/1 -> Cos8/1
  Subtract1/1 -> Divide/2
  Sin/1 -> Multiply/2
  deg2rad2/1 -> Cos3/1
  Sin3/1 -> Multiply10/2
  Constant10/1 -> Subtract1/1
  Sum5/1 -> Minus4/1, Minus5/1  "Direction of Lon Track"
  Constant13/1 -> Switch3/3
  Saturation/1 -> Sim.Zpos/1  "Sim.Zpos"
  Multiply2/1 -> Sum2/2  "EastVelocity2LateralVelocity"
  Constant5/1 -> Switch1/3
  East1/1 -> Minus5/2
  Minus4/1 -> deg2rad6/1
  Sum8/1 -> Sim.Xpos/1, Sum10/1, Compare To Constant1/1, Subtract/1  "Sim.Xpos"
  Sum2/1 -> Sim.Vy/1  "Sim.Vy"
  Switch2/1 -> ?
  East/1 -> Minus1/2
  Cos7/1 -> Multiply5/1
  Cos1/1 -> Multiply7/1
  Minus7/1 -> deg2rad7/1
  Constant7/1 -> Sin/1
  deg2rad3/1 -> Cos2/1
  North1/1 -> Minus4/2
  Cos6/1 -> Multiply4/1
  deg2rad1/1 -> Cos1/1
  Cos4/1 -> Multiply1/1
  "East "/1 -> Minus3/2
  Minus6/1 -> deg2rad8/1
  deg2rad7/1 -> Cos6/1
  deg2rad5/1 -> Cos5/1
  Constant2/1 -> Sum3/2
  Cos5/1 -> Multiply8/1
  Constant4/1 -> Sum6/2
  Cos8/1 -> Multiply3/1
  Constant3/1 -> Sum5/2
  East 1/1 -> Minus7/2
  Constant11/1 -> Sin1/1
  Sin1/1 -> Divide/1
  Multiply9/1 -> Subtract2/1
  Minus1/1 -> deg2rad1/1
  Subtract2/1 -> Switch2/1
  Constant8/1 -> Sin2/1
  deg2rad6/1 -> Cos7/1
  Divide/1 -> Add/1
  Saturation1/1 -> Sim.Vz/1  "Sim.Vz"
  VGround_mps/1 -> Gain/1
  Sum7/1 -> Sim.Ypos/1  "Sim.Ypos"

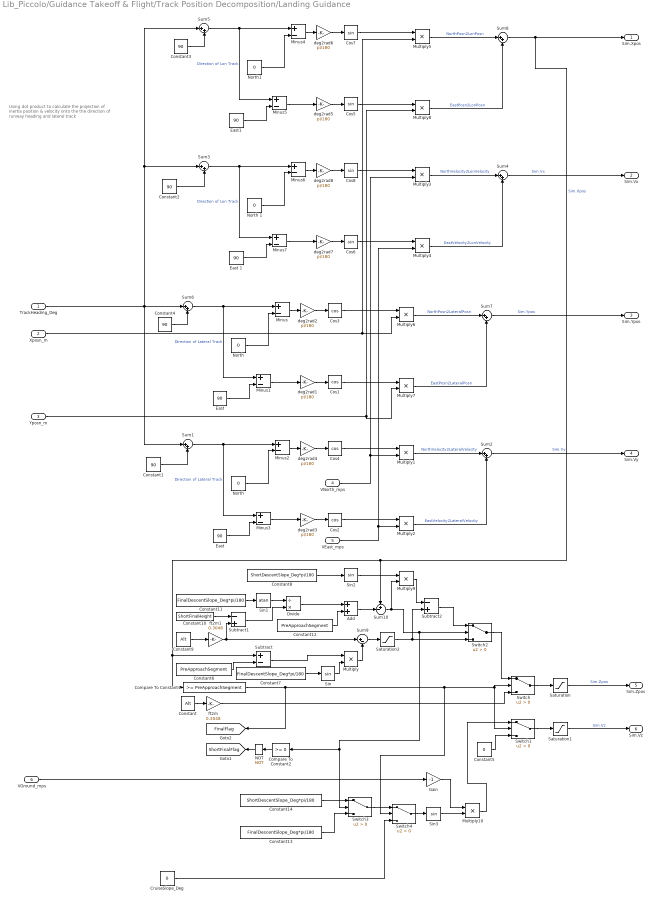
== system Lib_Piccolo/Guidance Takeoff & Flight/Track Position Decomposition/Landing Guidance ==
  note: Using dot product to calculate the projection of inertia position & velocity onto the
      | the direction of runway heading and lateral track
  TrackHeading_Deg : Inport
  Xposn_m : Inport  Port=2
  Yposn_m : Inport  Port=3
  VNorth_mps : Inport  Port=4
  VEast_mps : Inport  Port=5
  VGround_mps : Inport  Port=6
  Add : Sum
  Compare To Constant1 : simulink/Logic and Bit Operations/Compare To Constant  relop=>=  const=PreApproachSegment  OutDataTypeStr=uint8
  Compare To Constant2 : simulink/Logic and Bit Operations/Compare To Constant  relop=>=  const=0  OutDataTypeStr=uint8
  Constant : Constant  Value=Alt
  Constant{1..4} (4 alike) : Constant  Value=90
  Constant10 : Constant  Value=ShortFinalHeight
  Constant11 : Constant  Value=FinalDescentSlope_Deg*pi/180
  Constant12 : Constant  Value=PreApproachSegment
  Constant13 : Constant  Value=FinalDescentSlope_Deg*pi/180
  Constant14 : Constant  Value=ShortDescentSlope_Deg*pi/180
  Constant5 : Constant  Value=0
  Constant6 : Constant  Value=PreApproachSegment
  Constant7 : Constant  Value=FinalDescentSlope_Deg*pi/180
  Constant8 : Constant  Value=ShortDescentSlope_Deg*pi/180
  Constant9 : Constant  Value=Alt
  Cos{1..4} (4 alike) : Trigonometry  Operator=cos
  Cos{5..8} (4 alike) : Trigonometry
  CruiseSlope_Deg : Constant  Value=0
  Divide : Product  Inputs=/*
  East : Constant  Value=90
  "East " : Constant  Value=90
  East 1 : Constant  Value=90
  East1 : Constant  Value=90
  Gain : Gain  Gain=-1
  Minus{,1..7} (8 alike) : Sum  Inputs=+-
  Multiply{,1..10} (11 alike) : Product
  NOT : Logic  Operator=NOT  IconShape=distinctive  AllPortsSameDT=off  OutDataTypeStr=boolean
  North : Constant  Value=0
  "North " : Constant  Value=0
  North 1 : Constant  Value=0
  North1 : Constant  Value=0
  Saturation : Saturate  UpperLimit=AltMax  LowerLimit=TerrainHeight*0.3048
  Saturation1 : Saturate  UpperLimit=100  LowerLimit=-100
  Saturation2 : Saturate  UpperLimit=AltMax  LowerLimit=ShortFinalHeight
  Sin : Trigonometry
  Sin1 : Trigonometry  Operator=atan
  Sin2 : Trigonometry
  Sin3 : Trigonometry
  Subtract : Sum  Inputs=+-
  Subtract1 : Sum  Inputs=-+
  Subtract2 : Sum  Inputs=-+
  Sum{1..8} (8 alike) : Sum  Inputs=|++
  Sum10 : Sum  Inputs=+-|
  Sum9 : Sum  Inputs=|+-
  Switch{,1..4} (5 alike) : Switch  Criteria=u2 > Threshold
  deg2rad{1..8} (8 alike) : Gain  Gain=pi/180
  ft2m : Gain  Gain=0.3048
  ft2m1 : Gain  Gain=0.3048
  Sim.Xpos : Outport
  Sim.Vx : Outport  Port=2
  Sim.Ypos : Outport  Port=3
  Sim.Vy : Outport  Port=4
  Sim.Zpos : Outport  Port=5
  Sim.Vz : Outport  Port=6
  tag scope: FinalFlag=global, ShortFinalFlag=global
  wires:
  Multiply4/1 -> Sum4/2  "EastVelocity2LonVelocity"
  VNorth_mps/1 -> Multiply3/2, Multiply1/2
  Cos2/1 -> Multiply2/1
  Constant14/1 -> Switch3/1
  Switch4/1 -> Sin3/1
  Constant9/1 -> ft2m1/1
  Minus/1 -> deg2rad2/1
  Constant6/1 -> Subtract/2
  Add/1 -> Sum10/2
  Sum9/1 -> Saturation2/1
  Cos3/1 -> Multiply6/1
  Sum4/1 -> Sim.Vx/1  "Sim.Vx"
  Sum1/1 -> Minus2/1, Minus3/1  "Direction of Lateral Track"
  deg2rad4/1 -> Cos4/1
  Sum6/1 -> Minus/1, Minus1/1  "Direction of Lateral Track"
  Constant12/1 -> Add/2
  Minus5/1 -> deg2rad5/1
  VEast_mps/1 -> Multiply4/2, Multiply2/2
  Sum10/1 -> Switch3/2, Compare To Constant2/1, Switch2/2, Multiply9/2
  Gain/1 -> Multiply10/1
  North/1 -> Minus/2
  Sum3/1 -> Minus6/1, Minus7/1  "Direction of Lon Track"
  Minus3/1 -> deg2rad3/1
  CruiseSlope_Deg/1 -> Switch4/3
  TrackHeading_Deg/1 -> Sum6/1, Sum3/1, Sum5/1, Sum1/1
  Multiply10/1 -> Switch1/1
  Multiply5/1 -> Sum8/1  "NorthPosn2LonPosn"
  Saturation2/1 -> Subtract2/2, Switch2/3
  Multiply7/1 -> Sum7/2  "EastPosn2LateralPosn"
  ft2m/1 -> Switch/3
  Multiply8/1 -> Sum8/2  "EastPosn2LonPosn"
  Minus2/1 -> deg2rad4/1
  Xposn_m/1 -> Multiply5/2, Multiply6/2
  Multiply6/1 -> Sum7/1  "NorthPosn2LateralPosn"
  Multiply/1 -> Sum9/2
  Multiply1/1 -> Sum2/1  "NorthVelocity2LateralVelocity"
  Sin2/1 -> Multiply9/1
  Constant1/1 -> Sum1/2
  NOT/1 -> [ShortFinalFlag]
  Compare To Constant1/1 -> Switch4/2, Switch/2, Switch1/2, [FinalFlag]
  "North "/1 -> Minus2/2
  Multiply3/1 -> Sum4/1  "NorthVelocity2LonVelocity"
  Switch1/1 -> Saturation1/1
  Yposn_m/1 -> Multiply7/2, Multiply8/2
  Switch/1 -> Saturation/1
  ft2m1/1 -> Subtract1/2, Sum9/1
  Switch3/1 -> Switch4/1
  North 1/1 -> Minus6/2
  Subtract/1 -> Multiply/1
  Compare To Constant2/1 -> NOT/1
  deg2rad8/1 -> Cos8/1
  Subtract1/1 -> Divide/2
  Sin/1 -> Multiply/2
  deg2rad2/1 -> Cos3/1
  Sin3/1 -> Multiply10/2
  Constant10/1 -> Subtract1/1
  Sum5/1 -> Minus4/1, Minus5/1  "Direction of Lon Track"
  Constant13/1 -> Switch3/3
  Constant/1 -> ft2m/1
  Saturation/1 -> Sim.Zpos/1  "Sim.Zpos"
  Multiply2/1 -> Sum2/2  "EastVelocity2LateralVelocity"
  Constant5/1 -> Switch1/3
  East1/1 -> Minus5/2
  Minus4/1 -> deg2rad6/1
  Sum8/1 -> Sim.Xpos/1, Sum10/1, Compare To Constant1/1, Subtract/1  "Sim.Xpos"
  Sum2/1 -> Sim.Vy/1  "Sim.Vy"
  Switch2/1 -> Switch/1
  East/1 -> Minus1/2
  Cos7/1 -> Multiply5/1
  Cos1/1 -> Multiply7/1
  Minus7/1 -> deg2rad7/1
  Constant7/1 -> Sin/1
  deg2rad3/1 -> Cos2/1
  North1/1 -> Minus4/2
  Cos6/1 -> Multiply4/1
  deg2rad1/1 -> Cos1/1
  Cos4/1 -> Multiply1/1
  "East "/1 -> Minus3/2
  Minus6/1 -> deg2rad8/1
  deg2rad7/1 -> Cos6/1
  deg2rad5/1 -> Cos5/1
  Constant2/1 -> Sum3/2
  Cos5/1 -> Multiply8/1
  Constant4/1 -> Sum6/2
  Cos8/1 -> Multiply3/1
  Constant3/1 -> Sum5/2
  East 1/1 -> Minus7/2
  Constant11/1 -> Sin1/1
  Sin1/1 -> Divide/1
  Multiply9/1 -> Subtract2/1
  Minus1/1 -> deg2rad1/1
  Subtract2/1 -> Switch2/1
  Constant8/1 -> Sin2/1
  deg2rad6/1 -> Cos7/1
  Divide/1 -> Add/1
  Saturation1/1 -> Sim.Vz/1  "Sim.Vz"
  VGround_mps/1 -> Gain/1
  Sum7/1 -> Sim.Ypos/1  "Sim.Ypos"

== system Lib_Piccolo/Piccolo State Machine/Flight State Machine/Abort Logic ==
  note: Cross-track abort logic - this is a Piccolo feature.
  note: "User" abort logic to trigger RTO at given speed. This is not a Piccolo feature but useful for testing RTO conditions.
      |
      | Currently triggering off IAS only, but can use ground speed or other sources.
  IAS : Inport
  GroundSpeed : Inport  Port=2
  AND2 : Logic  IconShape=distinctive  AllPortsSameDT=off  OutDataTypeStr=boolean
  AND3 : Logic  IconShape=distinctive  AllPortsSameDT=off  OutDataTypeStr=boolean
  Compare To Constant5 : simulink/Logic and Bit Operations/Compare To Constant  relop=>=  const=RTO_Speed  OutDataTypeStr=boolean
  Compare To Constant6 : simulink/Logic and Bit Operations/Compare To Constant  relop=>  const=0  OutDataTypeStr=boolean
  Constant : Constant
  Constant7 : Constant  Value=EnableCrossTrackAbort
  Constant8 : Constant  Value=RTO_Speed
  Latch : $bdroot/Latch  SystemSampleTime=-1
  OR : Logic  Operator=OR  IconShape=distinctive  AllPortsSameDT=off  OutDataTypeStr=boolean
  Terminator : Terminator
  Flag_TakeoffAbort : Outport
  wires:
  AND2/1 -> OR/1
  IAS/1 -> Compare To Constant5/1
  Constant7/1 -> AND2/1
  Constant8/1 -> Compare To Constant6/1
  [Flag_CrossTrackAbort] -> AND2/2
  Compare To Constant6/1 -> AND3/1
  OR/1 -> Latch/1
  AND3/1 -> OR/2  "Flag_UserRTO"
  GroundSpeed/1 -> Terminator/1
  Compare To Constant5/1 -> AND3/2
  Latch/1 -> Flag_TakeoffAbort/1  "Flag_TakeoffAbort"
  Constant/1 -> Latch/2

== system Lib_Piccolo/Piccolo State Machine/Flight State Machine/Latch ==
  D : Inport
  Enable/!Rst : Inport  Port=2
  AND : Logic  IconShape=distinctive  AllPortsSameDT=off  OutDataTypeStr=boolean
  Constant : Constant
  OR : Logic  Operator=OR  IconShape=distinctive  AllPortsSameDT=off  OutDataTypeStr=boolean
  Switch : Switch  Criteria=u2 > Threshold  Threshold=0.5
  Unit Delay : UnitDelay  SampleTime=-1
  Q_Latched : Outport
  wires:
  Unit Delay/1 -> OR/2
  Switch/1 -> Q_Latched/1, Unit Delay/1
  D/1 -> Switch/3, OR/1
  OR/1 -> AND/1
  AND/1 -> Switch/2
  Enable/!Rst/1 -> AND/2
  Constant/1 -> Switch/1

== system Lib_Piccolo/Piccolo State Machine/Flight State Machine/Latch1 ==
  D : Inport
  Enable/!Rst : Inport  Port=2
  AND : Logic  IconShape=distinctive  AllPortsSameDT=off  OutDataTypeStr=boolean
  Constant : Constant
  OR : Logic  Operator=OR  IconShape=distinctive  AllPortsSameDT=off  OutDataTypeStr=boolean
  Switch : Switch  Criteria=u2 > Threshold  Threshold=0.5
  Unit Delay : UnitDelay  SampleTime=-1
  Q_Latched : Outport
  wires:
  Unit Delay/1 -> OR/2
  Switch/1 -> Q_Latched/1, Unit Delay/1
  D/1 -> Switch/3, OR/1
  OR/1 -> AND/1
  AND/1 -> Switch/2
  Enable/!Rst/1 -> AND/2
  Constant/1 -> Switch/1

== system Lib_Piccolo/Piccolo State Machine/Flight State Machine/Latch2 ==
  D : Inport
  Enable/!Rst : Inport  Port=2
  AND : Logic  IconShape=distinctive  AllPortsSameDT=off  OutDataTypeStr=boolean
  Constant : Constant
  OR : Logic  Operator=OR  IconShape=distinctive  AllPortsSameDT=off  OutDataTypeStr=boolean
  Switch : Switch  Criteria=u2 > Threshold  Threshold=0.5
  Unit Delay : UnitDelay  SampleTime=-1
  Q_Latched : Outport
  wires:
  Unit Delay/1 -> OR/2
  Switch/1 -> Q_Latched/1, Unit Delay/1
  D/1 -> Switch/3, OR/1
  OR/1 -> AND/1
  AND/1 -> Switch/2
  Enable/!Rst/1 -> AND/2
  Constant/1 -> Switch/1

== system Lib_Piccolo/Piccolo State Machine/Flight State Machine/Timer ==
  Run/!Reset : Inport
  Compare To Constant1 : simulink/Logic and Bit Operations/Compare To Constant  relop=>  const=0  OutDataTypeStr=uint8
  Compare To Constant3 : simulink/Logic and Bit Operations/Compare To Constant  relop===  const=0  OutDataTypeStr=boolean
  Discrete-Time Integrator : DiscreteIntegrator  ExternalReset=level  SampleTime=-1  OutDataTypeStr=double  ICPrevOutput=DiscIntNeverNeededParam  ICPrevScaledInput=DiscIntNeverNeededParam
  timeOut_s : Outport
  wires:
  Compare To Constant3/1 -> Discrete-Time Integrator/2
  Run/!Reset/1 -> Compare To Constant3/1, Compare To Constant1/1
  Discrete-Time Integrator/1 -> timeOut_s/1
  Compare To Constant1/1 -> Discrete-Time Integrator/1

== system Lib_Piccolo/Piccolo State Machine/Landing State Machine/Flare Detection ==
  Compare To Constant : simulink/Logic and Bit Operations/Compare To Constant  relop=>  const=0  OutDataTypeStr=boolean
  Delay : Delay  DelayLength=0.04/dt  InitialCondition=Alt*0.3048
  "FlareHeight_m " : Constant  Value=FlareHeight
  Sum : Sum  Inputs=|++
  Sum1 : Sum  Inputs=|+-
  Sum2 : Sum  Inputs=|++
  Sum4 : Sum  Inputs=|+-
  Sum5 : Sum  Inputs=|+-
  Terminator10 : Terminator
  "TerrainHeight " : Constant  Value=TerrainHeight
  VehicleRestingHeight : Constant  Value=DesktopSimTerrainOffset_m
  ft to m : Gain  Gain=0.3048
  tag scope: AltAGL_m=global, FlareFlag=global
  wires:
  Sum2/1 -> Sum1/2
  Sum1/1 -> Compare To Constant/1, [FlareFlag]
  VehicleRestingHeight/1 -> Sum2/2, Sum5/2
  ft to m/1 -> Sum4/2, Sum/1
  "TerrainHeight "/1 -> ft to m/1
  Sum5/1 -> [AltAGL_m]  "AltAGL_m"
  Sum4/1 -> Sum5/1
  Compare To Constant/1 -> Terminator10/1  "Sim.FlareFlag"
  "FlareHeight_m "/1 -> Sum/2
  [Alt_m] -> Delay/1, Sum4/1
  Delay/1 -> Sum1/1
  Sum/1 -> Sum2/1

== system Lib_Piccolo/Piccolo State Machine/Landing State Machine/FlareLatch ==
  apMode : Inport
  FlareFlag : Inport  Port=2
  Compare To Constant1 : simulink/Logic and Bit Operations/Compare To Constant  relop=>=  const=6  OutDataTypeStr=boolean
  Compare To Constant2 : simulink/Logic and Bit Operations/Compare To Constant  relop=<  const=0  OutDataTypeStr=boolean
  Latch : Subsystem
  NOT3 : Logic  Operator=NOT  IconShape=distinctive  AllPortsSameDT=off  OutDataTypeStr=boolean
  OR : Logic  Operator=OR  IconShape=distinctive  AllPortsSameDT=off  OutDataTypeStr=boolean
  Unit Delay : UnitDelay  SampleTime=-1
  FlareLatch : Outport
  wires:
  Compare To Constant2/1 -> OR/1, Latch/1(D)
  OR/1 -> NOT3/1
  FlareFlag/1 -> Compare To Constant2/1
  Latch/1(Q_Latched) -> OR/2
  NOT3/1 -> FlareLatch/1
  apMode/1 -> Unit Delay/1
  Compare To Constant1/1 -> Latch/2(Enable/!Rst)
  Unit Delay/1 -> Compare To Constant1/1

== system Lib_Piccolo/Piccolo State Machine/Landing State Machine/ShortFinal Detection ==
  Compare To Constant4 : simulink/Logic and Bit Operations/Compare To Constant  relop=>  const=0  OutDataTypeStr=boolean
  ShortFinalHeight : Constant  Value=ShortFinalHeight
  Sum3 : Sum  Inputs=|+-
  tag scope: ShortFinalFlag=global
  wires:
  Compare To Constant4/1 -> [ShortFinalFlag]  "Sim.ShortFinalFlag"
  ShortFinalHeight/1 -> Sum3/2
  [Alt_m] -> Sum3/1
  Sum3/1 -> Compare To Constant4/1

== system Lib_Piccolo/Piccolo State Machine LDG/FlareLatch/Latch ==
  D : Inport
  Enable/!Rst : Inport  Port=2
  AND : Logic  IconShape=distinctive  AllPortsSameDT=off  OutDataTypeStr=boolean
  Constant : Constant
  OR : Logic  Operator=OR  IconShape=distinctive  AllPortsSameDT=off  OutDataTypeStr=boolean
  Switch : Switch  Criteria=u2 > Threshold  Threshold=0.5
  Unit Delay : UnitDelay  SampleTime=-1
  Q_Latched : Outport
  wires:
  Unit Delay/1 -> OR/2
  Switch/1 -> Q_Latched/1, Unit Delay/1
  D/1 -> Switch/3, OR/1
  OR/1 -> AND/1
  AND/1 -> Switch/2
  Enable/!Rst/1 -> AND/2
  Constant/1 -> Switch/1
